simulink model "Lab2_Task_1"  (R2025a)
settings: Solver=FixedStepAuto  StartTime=0.0  StopTime=inf  RelTol=1e-3
model workspace (MAT data in the model file):
  SL_ROS_VariableLengthArrays_MaxSizes.CommonInfo.ArrayTruncateAction = 'EmitWarning'
  SL_ROS_VariableLengthArrays_MaxSizes.MsgTypeMap = containers.Map
  SL_ROS_VariableLengthArrays_MaxSizes.MsgTypeMap.serialization.keys = {'sensor_msgs/LaserScan'}
  SL_ROS_VariableLengthArrays_MaxSizes.MsgTypeMap.serialization.values{1}(1).PropertyName = 'intensities'
  SL_ROS_VariableLengthArrays_MaxSizes.MsgTypeMap.serialization.values{1}(1).DataType = 'single'
  SL_ROS_VariableLengthArrays_MaxSizes.MsgTypeMap.serialization.values{1}(1).MaxLength = 360
  SL_ROS_VariableLengthArrays_MaxSizes.MsgTypeMap.serialization.values{1}(2).PropertyName = 'ranges'
  SL_ROS_VariableLengthArrays_MaxSizes.MsgTypeMap.serialization.values{1}(2).DataType = 'single'
  SL_ROS_VariableLengthArrays_MaxSizes.MsgTypeMap.serialization.values{1}(2).MaxLength = 360
  SL_ROS_VariableLengthArrays_MaxSizes.MsgTypeMap.serialization.uniformity = 0
  SL_ROS_VariableLengthArrays_MaxSizes.MsgTypeMap.serialization.keyType = 'char'
  SL_ROS_VariableLengthArrays_MaxSizes.MsgTypeMap.serialization.valueType = 'any'
undefined symbols (not defined in the file or in its folder): header, twist
libraries: ros2lib x4, simulink x2
settings Model: Creator=scott  LastModifiedBy=david
settings OptimizationCC: DefaultParameterBehavior=Inlined  EnhancedBackFolding=on  PassReuseOutputArgsAs=Individual arguments  ZeroExternalMemoryAtStartup=off  ZeroInternalMemoryAtStartup=off  MaxStackSize=64  OptimizeBlockOrder=speed  DifferentSizesBufferReuse=on  OptimizationCustomize=off  EfficientTunableParamExpr=on
settings DebuggingCC: ParameterTunabilityLossMsg=error
settings HardwareCC: ProdBitPerPointer=32.0  ProdBitPerSizeT=32.0  ProdBitPerPtrDiffT=32.0  ProdWordSize=32.0  ProdHWDeviceType=Intel->x86-32 (Windows32)  UseEmbeddedCoderFeatures=off
settings SFSimCC: MATLABDynamicMemAlloc=off
settings RTWCC: SystemTargetFile=ert.tlc  HardwareBoard=Robot Operating System 2 (ROS 2)  TLCOptions="-aInlineSetEventsForThisBaseRateFcn=TLC_FALSE -aSuppressMultiTaskScheduler=TLC_FALSE  -aRateBasedStepFcn=0"  TemplateMakefile=ert_default_tmf  Toolchain=Colcon Tools  TargetLang=C++  Description=Embedded Coder
settings CodeAppCC: ForceParamTrailComments=on  IgnoreCustomStorageClasses=off  OperatorAnnotations=on  SimulinkDataObjDesc=on  SFDataObjDesc=on  InsertBlockDesc=on
settings ERTTargetCC: ExtModeTransport=2.0  ExtModeAutomaticAllocSize=off  RootIOFormat=Structure reference  CodeInterfacePackaging=C++ class  SupportNonInlinedSFcns=on

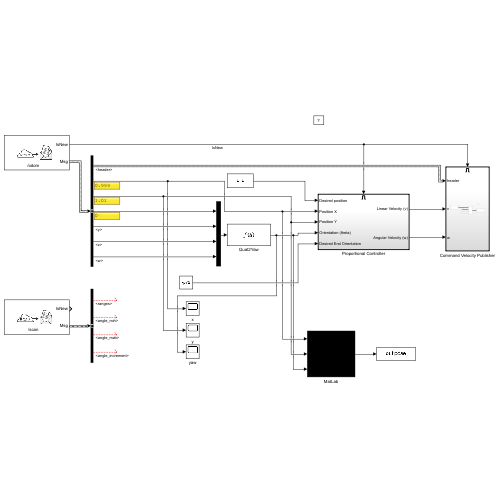
[thumbnail: Simulink's stored preview of the top-level diagram]
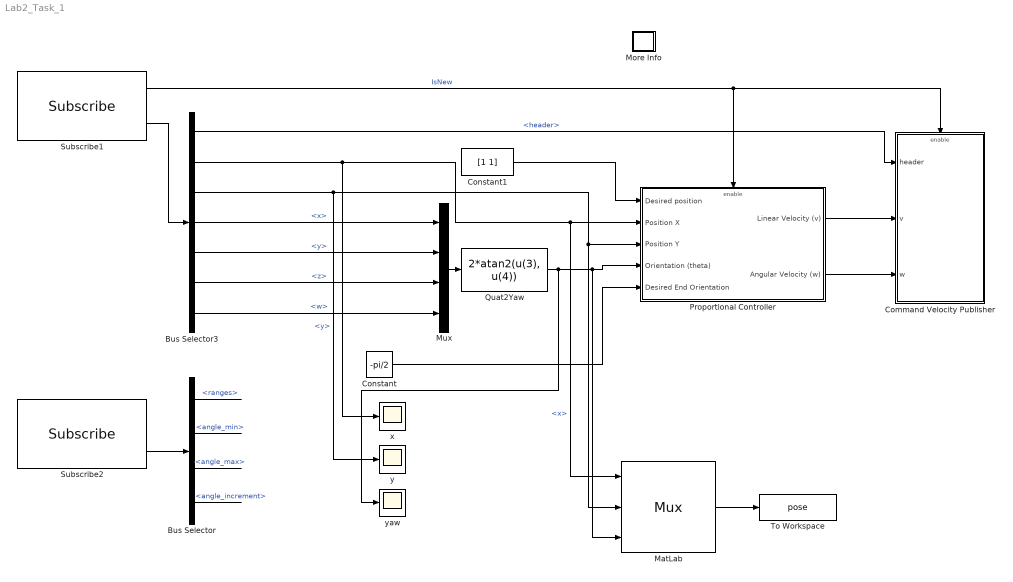
== system Lab2_Task_1 ==
  Bus Selector : BusSelector  OutputSignals=ranges,angle_min,angle_max,angle_increment
  Bus Selector3 : BusSelector  OutputSignals=header,pose.pose.position.x,pose.pose.position.y,pose.pose.orientation.x,pose.pose.orientation.y,pose.pose.orientation.z,pose.pose.orientation.w
  Command Velocity Publisher : Subsystem
  Constant : Constant  Value=-pi/2
  Constant1 : Constant  Value=[1 1]
  MatLab : Mux  Inputs=3
  More Info : Subsystem
      settings: OpenFcn=showdemo(bdroot(gcb))
      mask Display: disp('?')
  Mux : Mux
  Proportional Controller : Subsystem
  Quat2Yaw : Fcn  Expr=2*atan2(u(3), u(4))
  Subscribe1 : ros2lib/Subscribe  topicSource=Select from ROS network  topic=/odom  messageType=nav_msgs/Odometry  sampleTime=-1  QOSHistory=Keep last  QOSDepth=10  QOSReliability=Reliable  QOSDurability=Volatile  QOSDeadline=Inf  QOSLifespan=Inf  QOSLiveliness=Automatic  QOSLeaseDuration=Inf  QOSAvoidROSNamespaceConventions=off
  Subscribe2 : ros2lib/Subscribe  topicSource=Select from ROS network  topic=/scan  messageType=sensor_msgs/LaserScan  sampleTime=-1  QOSHistory=Keep last  QOSDepth=10  QOSReliability=Best effort  QOSDurability=Volatile  QOSDeadline=Inf  QOSLifespan=Inf  QOSLiveliness=Automatic  QOSLeaseDuration=Inf  QOSAvoidROSNamespaceConventions=off
  To Workspace : ToWorkspace  VariableName=pose  SaveFormat=Timeseries  SampleTime=-1
  x : Scope
      settings: ActiveDisplayYMinimum=-0.12491854268567354  ActiveDisplayYMaximum=1.1242668841708461
  y : Scope
      settings: ActiveDisplayYMinimum=-0.14797806498971205  ActiveDisplayYMaximum=1.3318025599545946  DataLoggingVariableName=ScopeData2
  yaw : Scope
      settings: ActiveDisplayYMinimum=-6.2239731252193451  ActiveDisplayYMaximum=1.5603109300136566  DataLoggingVariableName=ScopeData3
  wires:
  Subscribe1/2 -> Bus Selector3/1
  Subscribe1/1 -> Command Velocity Publisher/Enable, Proportional Controller/Enable  "IsNew"
  Proportional Controller/1(Linear Velocity (v)) -> Command Velocity Publisher/2(v)
  Proportional Controller/2(Angular Velocity (w)) -> Command Velocity Publisher/3(w)
  Bus Selector3/1 -> Command Velocity Publisher/1(header)  "<header>"
  Bus Selector3/2 -> x/1, MatLab/1, Proportional Controller/2(Position X)  "<x>"
  Bus Selector3/3 -> y/1, MatLab/2, Proportional Controller/3(Position Y)  "<y>"
  Bus Selector3/4 -> Mux/1  "<x>"
  Bus Selector3/5 -> Mux/2  "<y>"
  Bus Selector3/6 -> Mux/3  "<z>"
  Bus Selector3/7 -> Mux/4  "<w>"
  Subscribe2/2 -> Bus Selector/1
  Bus Selector/1 -> ?  "<ranges>"
  Bus Selector/2 -> ?  "<angle_min>"
  Bus Selector/3 -> ?  "<angle_max>"
  Bus Selector/4 -> ?  "<angle_increment>"
  Mux/1 -> Quat2Yaw/1
  Quat2Yaw/1 -> yaw/1, MatLab/3, Proportional Controller/4(Orientation (theta))
  Constant/1 -> Proportional Controller/5(Desired End Orientation)
  Constant1/1 -> Proportional Controller/1(Desired position)
  MatLab/1 -> To Workspace/1

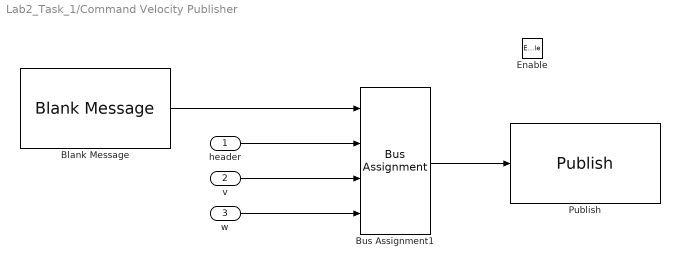
== system Lab2_Task_1/Command Velocity Publisher ==
  header : Inport
  v : Inport  Port=2
  w : Inport  Port=3
  Enable : EnablePort
  Blank Message : ros2lib/Blank Message  messageClass=Message  entityType=geometry_msgs/TwistStamped  messageType=geometry_msgs/TwistStamped  SampleTime=inf
  Bus Assignment1 : BusAssignment  DialogController=Simulink.DDGSource_BusAssignment  AssignedSignals=header,twist.linear.x,twist.angular.z
  Publish : ros2lib/Publish  topicSource=Select from ROS network  topic=/cmd_vel  messageType=geometry_msgs/TwistStamped  QOSHistory=Keep last  QOSDepth=10  QOSReliability=Reliable  QOSDurability=Volatile  QOSDeadline=Inf  QOSLifespan=Inf  QOSLiveliness=Automatic  QOSLeaseDuration=Inf  QOSAvoidROSNamespaceConventions=off
  wires:
  Bus Assignment1/1 -> Publish/1
  Blank Message/1 -> Bus Assignment1/1
  header/1 -> Bus Assignment1/2
  v/1 -> Bus Assignment1/3
  w/1 -> Bus Assignment1/4

== system Lab2_Task_1/More Info ==

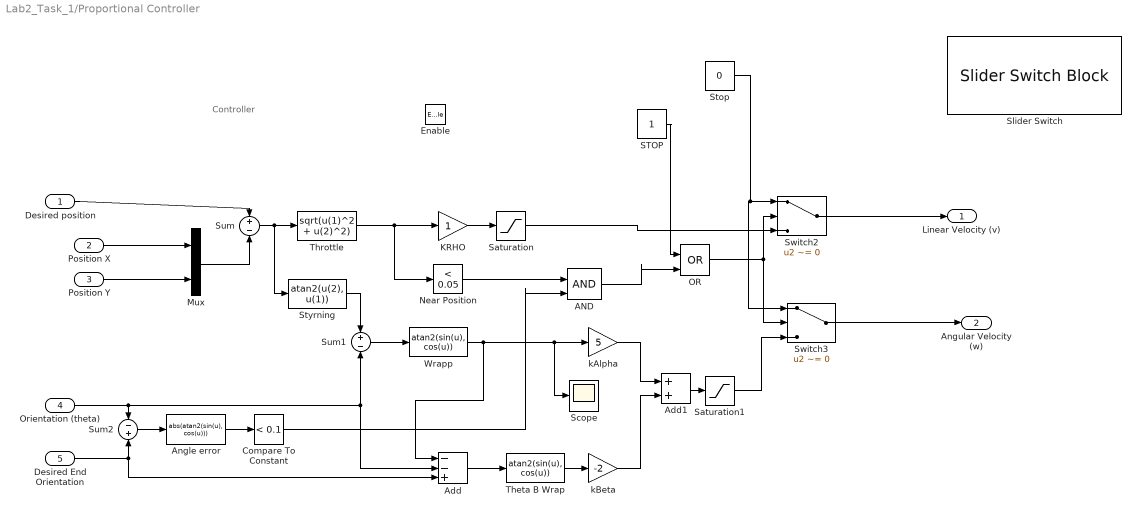
== system Lab2_Task_1/Proportional Controller ==
  note: Controller
  Desired position : Inport
  Position X : Inport  Port=2
  Position Y : Inport  Port=3
  Orientation (theta) : Inport  Port=4
  Desired End Orientation : Inport  Port=5
  Enable : EnablePort
  AND : Logic  IconShape=distinctive  AllPortsSameDT=off  OutDataTypeStr=boolean
  Add : Sum  Inputs=--+
  Add1 : Sum
  Angle error : Fcn  Expr=abs(atan2(sin(u), cos(u)))
  Compare To Constant : simulink/Logic and Bit Operations/Compare To Constant  relop=<  const=0.1  OutDataTypeStr=boolean
  KRHO : Gain
  Mux : Mux  Inputs=2
  Near Position : simulink/Logic and Bit Operations/Compare To Constant  relop=<  const=0.05  OutDataTypeStr=boolean
  OR : Logic  Operator=OR  IconShape=distinctive  AllPortsSameDT=off  OutDataTypeStr=boolean
  "STOP " : Constant
  Saturation : Saturate  UpperLimit=0.22
  Saturation1 : Saturate  UpperLimit=2.84  LowerLimit=-2.84
  Scope : Scope
      settings: ActiveDisplayYMinimum=-1  ActiveDisplayYMaximum=1
  Slider Switch : SliderSwitchBlock
  Stop : Constant  Value=0
  Styrning : Fcn  Expr=atan2(u(2), u(1))
  Sum : Sum  Inputs=+-
  Sum1 : Sum  Inputs=+-
  Sum2 : Sum  Inputs=-+
  Switch2 : Switch  Criteria=u2 ~= 0  SaturateOnIntegerOverflow=off  InputSameDT=off
  Switch3 : Switch  Criteria=u2 ~= 0  SaturateOnIntegerOverflow=off  InputSameDT=off
  Theta B Wrap : Fcn  Expr=atan2(sin(u), cos(u))
  Throttle : Fcn  Expr=sqrt(u(1)^2 + u(2)^2)
  Wrapp : Fcn  Expr=atan2(sin(u), cos(u))
  kAlpha : Gain  Gain=5
  kBeta : Gain  Gain=-2
  Linear Velocity (v) : Outport  VectorParamsAs1DForOutWhenUnconnected=off
  Angular Velocity (w) : Outport  Port=2  VectorParamsAs1DForOutWhenUnconnected=off
  wires:
  Stop/1 -> Switch3/1, Switch2/1
  "STOP "/1 -> OR/1
  Switch2/1 -> Linear Velocity (v)/1
  Switch3/1 -> Angular Velocity (w)/1
  Desired position/1 -> Sum/1
  Mux/1 -> Sum/2
  Throttle/1 -> Near Position/1, KRHO/1
  Sum/1 -> Styrning/1, Throttle/1
  Styrning/1 -> Sum1/1
  Orientation (theta)/1 -> Sum2/1, Add/2, Sum1/2
  Sum1/1 -> Wrapp/1
  Wrapp/1 -> Add/1, Scope/1, kAlpha/1
  Desired End Orientation/1 -> Sum2/2, Add/3
  Add/1 -> Theta B Wrap/1
  Theta B Wrap/1 -> kBeta/1
  kAlpha/1 -> Add1/1
  kBeta/1 -> Add1/2
  Add1/1 -> Saturation1/1
  KRHO/1 -> Saturation/1
  Position X/1 -> Mux/1
  Position Y/1 -> Mux/2
  Saturation/1 -> Switch2/3
  Saturation1/1 -> Switch3/3
  Sum2/1 -> Angle error/1
  Angle error/1 -> Compare To Constant/1
  Near Position/1 -> AND/1
  Compare To Constant/1 -> AND/2
  AND/1 -> OR/2
  OR/1 -> Switch2/2, Switch3/2
